simulink model "PV_twin_final"  (R2024b)
settings: Solver=ode23t  StartTime=0.0  StopTime=2  RelTol=1e-3
InitFcn:
  | Ts_Control = 10e-5;
  | Ts_Power = 80e-6;
  | Sensor_Ts = 1e-05;
libraries: spsSeriesRLCBranchLib x4, spsIGBTDiodeLib x4, spsCurrentMeasurementLib x2, spsVoltageMeasurementLib x2, spsACVoltageSourceLib x1, spsDiodeLib x1, spsIGBTLib x1, slpidlib x1, spsPVArrayLib x1, spsPWMGeneratorDCDCLib x1, simulink x1, spspowerguiLib x1
settings Model: SimulationMode=accelerator  Creator=Deependra  LastModifiedBy=Asus
settings DataIOCC: ReturnWorkspaceOutputs=off
settings DebuggingCC: UnconnectedInputMsg=warning  UnconnectedOutputMsg=warning  UnconnectedLineMsg=warning  ArithmeticOperatorsInVariantConditions=warning
settings ModelReferenceCC: EnableRefExpFcnMdlSchedulingChecks=on
settings SFSimCC: SimUseLocalCustomCode=off  CustomCodeUndefinedFunction=UseInterfaceOnly
settings RTWCC: RTWUseLocalCustomCode=off  GPUComputeCapability=3.5

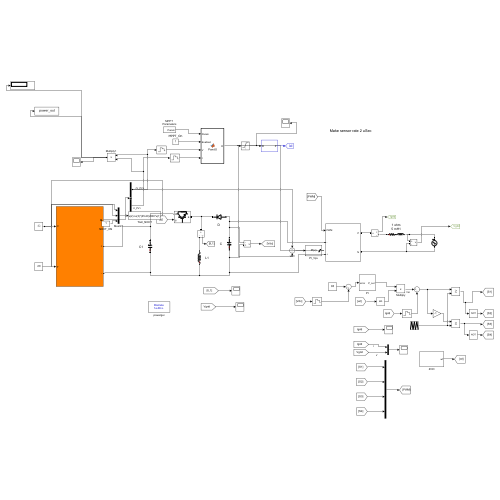
[thumbnail: Simulink's stored preview of the top-level diagram]
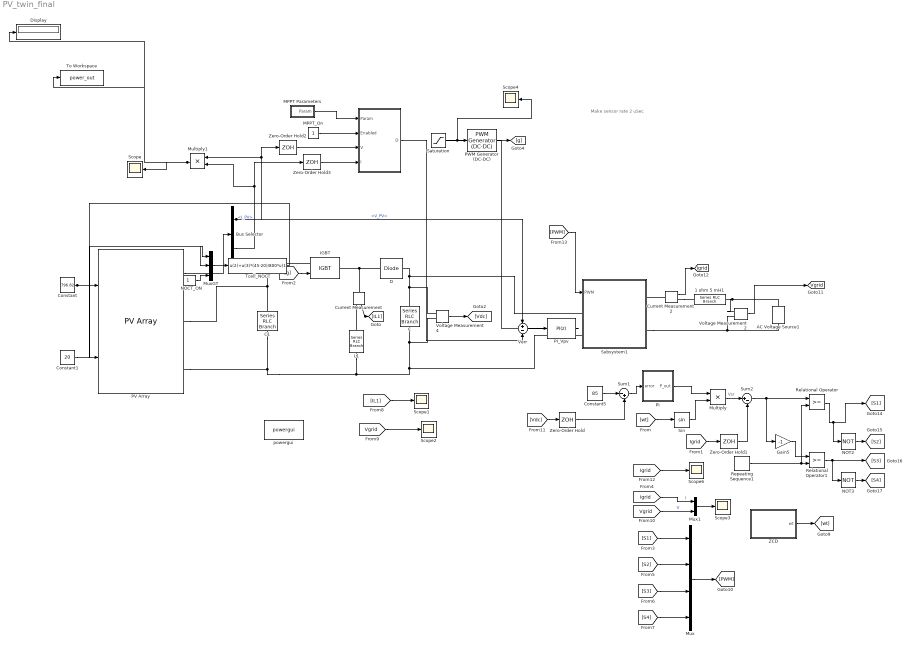
== system PV_twin_final ==
  note: Make sensor rate 2 uSec
  " " : MATLAB Function  TreatAsAtomicUnit=on
  1 ohm 5 mH1 : spsSeriesRLCBranchLib/Series RLC Branch  LConnTagsString=__new0  RConnTagsString=__new0  BranchType=RL  Resistance=1  Inductance=5e-3  SetiL0=off  InitialCurrent=0  Capacitance=400e-6  Setx0=off  InitialVoltage=0  Measurements=None
  AC Voltage Source1 : spsACVoltageSourceLib/AC Voltage Source  Amplitude=64  Phase=0  Frequency=50  SampleTime=0  Measurements=None  BusType=swing  Pref=10e3  Qref=0  Qmin=-inf  Qmax=+inf
  Bus Selector : BusSelector  OutputSignals=V_PV,I_PV
  C : spsSeriesRLCBranchLib/Series RLC Branch  LConnTagsString=__new0  RConnTagsString=__new0  BranchType=C  Resistance=1e-4  Inductance=200e-6  SetiL0=off  InitialCurrent=0  Capacitance=680e-6  Setx0=off  InitialVoltage=7.5  Measurements=None
  C1 : spsSeriesRLCBranchLib/Series RLC Branch  LConnTagsString=__new0  RConnTagsString=__new0  BranchType=C  Resistance=1e-4  Inductance=200e-6  SetiL0=off  InitialCurrent=0  Capacitance=680e-6  Setx0=off  InitialVoltage=7.5  Measurements=None
  Constant : Constant  Value=796.82
  Constant1 : Constant  Value=20
  Constant5 : Constant  Value=85
  Current Measurement : spsCurrentMeasurementLib/Current Measurement  PhasorSimulation=off  OutputType=Complex  PSBequivalent=0
  Current Measurement2 : spsCurrentMeasurementLib/Current Measurement  PhasorSimulation=off  OutputType=Complex  PSBequivalent=0
  "D " : spsDiodeLib/Diode  Ron=1e-3  Lon=0  Vf=0  IC=0  UseSnubber=off  Rs=inf  Cs=inf  Measurements=off
  Display : Display
  Gain5 : Gain  Gain=-1
  IGBT : spsIGBTLib/IGBT  Ron=0.000001  Lon=0  Vf=0  Tf=1e-6  Tt=2e-6  IC=0  Rs=1e5  Cs=inf  Measurements=off
  L1 : spsSeriesRLCBranchLib/Series RLC Branch  LConnTagsString=__new0  RConnTagsString=__new0  BranchType=L  Resistance=1e-4  Inductance=5e-3  SetiL0=off  InitialCurrent=14  Capacitance=30e-6  Setx0=off  InitialVoltage=150  Measurements=None
  MPPT Parameters : Subsystem
  MPPT_On : Constant
  Multiply : Product
  Multiply1 : Product
  Mux : Mux
  Mux1 : Mux  Inputs=2
  MuxGT : Mux  Inputs=3
  NOCT_ON : Constant
  NOT2 : Logic  Operator=NOT  AllPortsSameDT=off  OutDataTypeStr=boolean
  NOT3 : Logic  Operator=NOT  AllPortsSameDT=off  OutDataTypeStr=boolean
  PI : Subsystem
  PI_Vpv : slpidlib/PID Controller  Controller=PI  Form=Parallel  TimeDomain=Discrete-time  UseExternalTs=off  SampleTime=20e-6  IntegratorMethod=Forward Euler  FilterMethod=Forward Euler  ControllerParametersSource=internal  P=0.1  I=20  UseKiTs=off  D=0  UseExternalDerivativeSource=off  N=100  UseFilter=on  TunerSelectOption=Transfer Function Based (PID Tuner App)  InitialConditionSource=internal  InitialConditionForIntegrator=0.6  InitialConditionForFilter=0  DifferentiatorICPrevScaledInput=0  ExternalReset=none  TrackingMode=off  Kt=1  LimitOutput=on  SatLimitsSource=internal  UpperSaturationLimit=0.87  LowerSaturationLimit=0  LinearizeAsGain=off  AntiWindupMode=clamping  Kb=1  LimitIntegrator=off  UpperIntegratorSaturationLimit=inf  LowerIntegratorSaturationLimit=-inf  POutMin=[]  POutMax=[]  IOutMin=[]  IOutMax=[]  DOutMin=[]  DOutMax=[]  NOutMin=[]  NOutMax=[]  SumOutMin=[]  SumOutMax=[]  SaturationOutMin=[]  SaturationOutMax=[]  PParamMin=[]  PParamMax=[]  IParamMin=[]  IParamMax=[]  DParamMin=[]  DParamMax=[]  NParamMin=[]  NParamMax=[]  KbParamMin=[]  KbParamMax=[]  KtParamMin=[]  KtParamMax=[]  KbOutMin=[]  KbOutMax=[]  KtOutMin=[]  KtOutMax=[]  IntegratorOutMin=[]  IntegratorOutMax=[]  FilterOutMin=[]  FilterOutMax=[]  SumI1OutMin=[]  SumI1OutMax=[]  SumI2OutMin=[]  SumI2OutMax=[]  SumI3OutMin=[]  SumI3OutMax=[]  SumI4OutMin=[]  SumI4OutMax=[]  SumDOutMin=[]  SumDOutMax=[]  DifferentiatorOutMin=[]  DifferentiatorOutMax=[]  FilterDiffOutCoefMin=[]  FilterDiffOutCoefMax=[]  ReciprocalOutMin=[]  ReciprocalOutMax=[]  SumDenOutMin=[]  SumDenOutMax=[]  SumNumOutMin=[]  SumNumOutMax=[]  DivideOutMin=[]  DivideOutMax=[]  UdiffTsProdOutMin=[]  UdiffTsProdOutMax=[]  NTsProdOutMin=[]  NTsProdOutMax=[]  UintegralTsProdOutMin=[]  UintegralTsProdOutMax=[]  UngainTsProdOutMin=[]  UngainTsProdOutMax=[]  ClampingZeroOutDataTypeStr=Inherit: Inherit via back propagation  ClampingZeroOutMin=[]  ClampingZeroOutMax=[]  FilterDenConstantOutDataTypeStr=Inherit: Inherit via back propagation  FilterDenConstantOutMin=[]  FilterDenConstantOutMax=[]  PCopyOutDataTypeStr=Inherit: Inherit via back propagation  PCopyOutMin=[]  PCopyOutMax=[]  NCopyOutDataTypeStr=Inherit: Inherit via back propagation  NCopyOutMin=[]  NCopyOutMax=[]  IntegratorContinuousStateAttributes=''  IntegratorStateMustResolveToSignalObject=off  IntegratorRTWStateStorageClass=Auto  FilterContinuousStateAttributes=''  FilterStateMustResolveToSignalObject=off  FilterRTWStateStorageClass=Auto  ParallelPVariant=InternalParameters  IdealPVariant=Disabled  IVariant=InternalParameters  DVariant=Disabled  IntegratorVariant=Discrete  SatVariant=Enabled  AWVariant=DiscClampingParallel  PCopyVariant=Disabled  TRVariant=Disabled  FdbkBlocksVariant=Forward  IdealPFdbkVariant=Disabled  SatFdbkVariant=Disabled  DerivativeFilterVariant=Disabled  NVariant=Disabled  NCopyVariant=Disabled_SignalSpec  FilterICVariant=Disabled  IntegratorICVariant=InternalICs  ExternalResetVariant=Disabled  TRSumVariant=Passthrough  SumFdbkVariant=Disabled  SumVariant=Sum_PI  TsampFilterVariant=InternalTs  TsampNgainVariant=Passthrough  TsampIntegralVariant=Disabled_SignalSpec  ExternalSaturationOutDataTypeStr=Inherit: Same as second input  DerivativeSourceVariant=Disabled  PreIntVariant=InternalPreInt
      settings: LibrarySourceBlock=simulink/Discrete/Discrete PID Controller
  PV Array : spsPVArrayLib/PV Array  Npar=1  Nser=1  PlotType=one module @ 25 deg.C & specified irradiances  S_vec="[ 1000  500  100 ]"  Temp_C_vec="[ 45 25  ]"  ModuleName=User-defined  PlotWhenSelected=off  Pm=335.415  Ncell=72  Voc=46.27  Isc=9.41  Vm=37.9  Im=8.85  beta_Voc_pc=-0.30  alpha_Isc_pc=0.05  beta_Voc=-0.13881  alpha_Isc=0.004705  IL=9.4203  I0=3.2103e-11  nI=0.94785  Rsh=312.4283  Rs=0.34157  RobustModel=off  RobustCellTemperature=313.3991  BAL=off  Tc=1e-6  Tfilter=10e-5
  PWM Generator (DC-DC) : spsPWMGeneratorDCDCLib/PWM Generator (DC-DC)  Fsw=10e3  Ts=0
  Relational Operator : RelationalOperator  OutDataTypeStr=boolean  RndMeth=Simplest  InputSameDT=off
  Relational Operator1 : RelationalOperator  OutDataTypeStr=boolean  RndMeth=Simplest  InputSameDT=off
  Repeating Sequence1 : simulink/Sources/Repeating Sequence  rep_seq_t=[0 0.0001 0.0002]  rep_seq_y=[-1 1 -1]
  Saturation : Saturate  UpperLimit=0.87  LowerLimit=0
  Scope{,1..4,6} (6 alike) : Scope
  Sin : Trigonometry
  Subsystem1 : Subsystem
  Sum1 : Sum  Inputs=|-+
  Sum2 : Sum  Inputs=|+-
  Tcell_NOCT : Fcn  Expr=u(2)+u(3)*(45-20)/800*u(1)
  To Workspace : ToWorkspace  VariableName=power_out  SampleTime=-1
  Verr : Sum  Inputs=+-
  Voltage Measurement2 : spsVoltageMeasurementLib/Voltage Measurement  Tag=PoWeRsYsTeMmEaSuReMeNt  PhasorSimulation=off  OutputType=Magnitude  PSBequivalent=0
  Voltage Measurement4 : spsVoltageMeasurementLib/Voltage Measurement  PhasorSimulation=off  OutputType=Complex  PSBequivalent=0
  ZCD : Subsystem
  Zero-Order Hold : ZeroOrderHold  SampleTime=Sensor_Ts
  Zero-Order Hold1 : ZeroOrderHold  SampleTime=Sensor_Ts
  Zero-Order Hold2 : ZeroOrderHold  SampleTime=0.01
  Zero-Order Hold3 : ZeroOrderHold  SampleTime=0.01
  powergui : spspowerguiLib/powergui  Priority=1  SimulationMode=Discrete  SampleTime=1e-6  frequency=50  Iterations=50  frequencyindice=0  Pbase=100e6  ErrMax=1e-4  UnitsV=kV  UnitsW=MW  buscounter=0  FunctionMessages=off  echomessages=off  EnableUseOfTLC=off  CurrentSourceSwitches=off  DisableSnubberDevices=off  DisableRonSwitches=off  DisableVfSwitches=off  DisplayEquations=off  AutomaticDiscreteSolvers=off  SolverType=Tustin/Backward Euler (TBE)  Interpol=off  ExternalGateDelay=off  methode=off  Ts=100  x0status=blocks  SPID=on  SwTol=0  HookPort=off  NonlinearTolerance=1e-4  nMaxIteration=100  ContinueOnMaxIteration=off  RestoreLinks=warning  ResistiveCurrentMeasurement=off  Frange=[0:2:500]  Ylog=off  Xlog=on  ShowGrid=off  save=off  variable=ZData  structure=0  ZoomFFT=off  StartTime=0.0  cycles=1  DisplayStyle=1  fundamental=60  FreqAxis=off  MaxFrequency=1000  frequencyindicesteady=1  RmsSteady=1  display=off
  tag scope: Igrid=global, Vgrid=global
  wires:
  [g] -> IGBT/1
  Current Measurement/1 -> [IL1]
  Constant/1 -> PV Array/1, MuxGT/1
  PV Array/1 -> Bus Selector/1
  [Vdc] -> Zero-Order Hold/1
  Constant5/1 -> Sum1/1
  [wt] -> Sin/1
  Sin/1 -> Multiply/2
  Multiply/1 -> Sum2/1  "Vsr"
  [Igrid] -> Zero-Order Hold1/1
  ZCD/1(wt) -> [wt]
  [S2] -> Mux/2
  [S1] -> Mux/1
  [S3] -> Mux/3
  [S4] -> Mux/4
  Mux/1 -> [PWM]
  [IL1] -> Scope1/1
  [Vgrid] -> Scope2/1
  Voltage Measurement4/1 -> [Vdc]
  PWM Generator (DC-DC)/1 -> [g]
  MPPT_On/1 -> " "/2(Enabled)
  MPPT Parameters/1(Param) -> " "/1(Param)
  Bus Selector/1 -> Multiply1/1, Zero-Order Hold2/1, Verr/1  "<V_PV>"
  Bus Selector/2 -> Multiply1/2, Zero-Order Hold3/1  "<I_PV>"
  Saturation/1 -> Scope4/1, PWM Generator (DC-DC)/1
  Mux1/1 -> Scope3/1
  [Igrid] -> Mux1/1  "I"
  [Vgrid] -> Mux1/2  "V"
  Voltage Measurement2/1 -> [Vgrid]
  Current Measurement2/1 -> [Igrid]
  [PWM] -> Subsystem1/1(PWM)
  Relational Operator/1 -> NOT2/1, [S1]
  Repeating Sequence1/1 -> Relational Operator1/2, Relational Operator/2
  Relational Operator1/1 -> NOT3/1, [S3]
  NOT2/1 -> [S2]
  Sum2/1 -> Relational Operator/1, Gain5/1
  Gain5/1 -> Relational Operator1/1
  NOT3/1 -> [S4]
  [Igrid] -> Scope6/1
  Zero-Order Hold/1 -> Sum1/2
  Zero-Order Hold1/1 -> Sum2/2
  Sum1/1 -> PI/1(error)
  PI/1(P_out) -> Multiply/1
  Zero-Order Hold2/1 -> " "/3(V)
  Zero-Order Hold3/1 -> " "/4(I)
  Multiply1/1 -> Scope/1, To Workspace/1, Display/1
  " "/1(D) -> Verr/2
  Verr/1 -> PI_Vpv/1
  PI_Vpv/1 -> Saturation/1
  Constant1/1 -> MuxGT/2
  NOCT_ON/1 -> MuxGT/3
  MuxGT/1 -> Tcell_NOCT/1
  Tcell_NOCT/1 -> PV Array/2
  connections:
  C1/RConn1 -- PV Array/RConn1 -- IGBT/LConn1
  "D "/RConn1 -- Current Measurement/LConn1 -- IGBT/RConn1
  C/RConn1 -- Voltage Measurement4/LConn2 -- Subsystem1/LConn1 -- "D "/LConn1
  PV Array/RConn2 -- C1/LConn1 -- L1/LConn1 -- Subsystem1/LConn2 -- Voltage Measurement4/LConn1 -- C/LConn1
  L1/RConn1 -- Current Measurement/RConn1
  Voltage Measurement2/LConn1 -- 1 ohm 5 mH1/RConn1 -- AC Voltage Source1/RConn1
  Voltage Measurement2/LConn2 -- AC Voltage Source1/LConn1 -- Subsystem1/RConn2
  Current Measurement2/RConn1 -- 1 ohm 5 mH1/LConn1
  Current Measurement2/LConn1 -- Subsystem1/RConn1

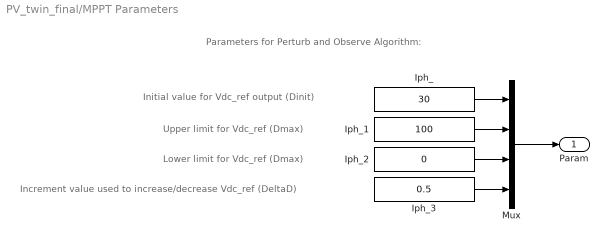
== system PV_twin_final/MPPT Parameters ==
  note: Parameters for Perturb and Observe Algorithm:
  note: Lower limit for Vdc_ref (Dmax)
  note: Initial value for Vdc_ref output (Dinit)
  note: Increment value used to increase/decrease Vdc_ref (DeltaD)
  note: Upper limit for Vdc_ref (Dmax)
  Iph_ : Constant  Value=30
  Iph_1 : Constant  Value=100
  Iph_2 : Constant  Value=0
  Iph_3 : Constant  Value=0.5
  Mux : Mux
  Param : Outport  VectorParamsAs1DForOutWhenUnconnected=off
  wires:
  Mux/1 -> Param/1
  Iph_3/1 -> Mux/4
  Iph_2/1 -> Mux/3
  Iph_1/1 -> Mux/2
  Iph_/1 -> Mux/1

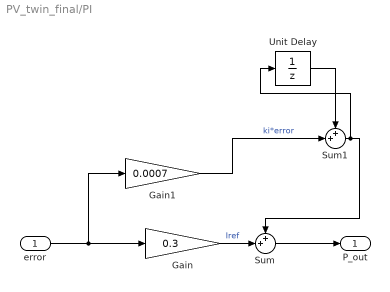
== system PV_twin_final/PI ==
  error : Inport
  Gain : Gain  Gain=0.3
  Gain1 : Gain  Gain=0.0007
  Sum : Sum  Inputs=++|
  Sum1 : Sum  Inputs=++|
  Unit Delay : UnitDelay  SampleTime=50e-6  HasFrameUpgradeWarning=on
  P_out : Outport  VectorParamsAs1DForOutWhenUnconnected=off
  wires:
  Gain/1 -> Sum/2  "Iref"
  error/1 -> Gain/1, Gain1/1
  Gain1/1 -> Sum1/2  "ki*error"
  Sum/1 -> P_out/1
  Unit Delay/1 -> Sum1/1
  Sum1/1 -> Sum/1, Unit Delay/1

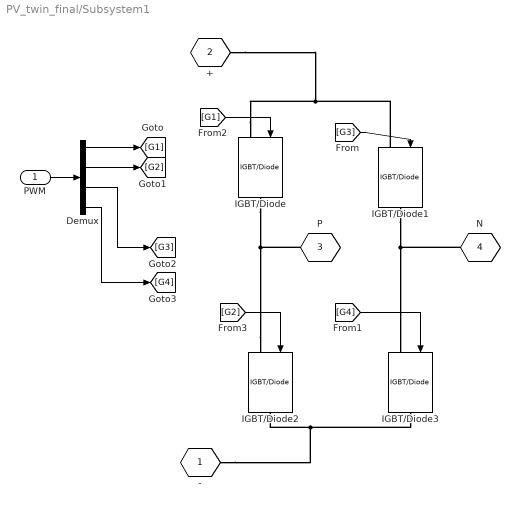
== system PV_twin_final/Subsystem1 ==
  PWM : Inport
  Demux : Demux
  IGBT/Diode{,1..3} (4 alike) : spsIGBTDiodeLib/IGBT//Diode  Ron=1e-3  Rs=1e5  Cs=inf  Measurements=off
  - : PMIOPort  Tag=PMCPort  Side=Left
  + : PMIOPort  Tag=PMCPort  Port=2  Side=Left
  "P " : PMIOPort  Tag=PMCPort  Port=3  Side=Right
  "N " : PMIOPort  Tag=PMCPort  Port=4  Side=Right
  wires:
  Demux/4 -> [G4]
  Demux/3 -> [G3]
  Demux/2 -> [G2]
  Demux/1 -> [G1]
  PWM/1 -> Demux/1
  [G4] -> IGBT/Diode3/1
  [G1] -> IGBT/Diode/1
  [G2] -> IGBT/Diode2/1
  [G3] -> IGBT/Diode1/1
  connections:
  IGBT/Diode/LConn1 -- +/RConn1 -- IGBT/Diode1/LConn1
  "N "/RConn1 -- IGBT/Diode3/LConn1 -- IGBT/Diode1/RConn1
  IGBT/Diode2/RConn1 -- -/RConn1 -- IGBT/Diode3/RConn1
  IGBT/Diode2/LConn1 -- "P "/RConn1 -- IGBT/Diode/RConn1

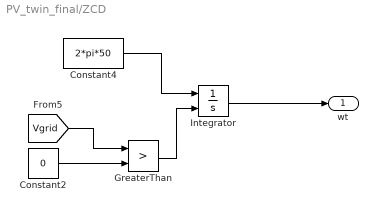
== system PV_twin_final/ZCD ==
  Constant2 : Constant  Value=0
  Constant4 : Constant  Value=2*pi*50
  GreaterThan : RelationalOperator  Operator=>  OutDataTypeStr=boolean  RndMeth=Simplest  InputSameDT=off
  Integrator : Integrator  ExternalReset=rising
  wt : Outport  VectorParamsAs1DForOutWhenUnconnected=off
  wires:
  Constant4/1 -> Integrator/1
  Integrator/1 -> wt/1
  [Vgrid] -> GreaterThan/1
  GreaterThan/1 -> Integrator/2
  Constant2/1 -> GreaterThan/2

== matlab function PV_twin_final/  ==
  settings: updateMethod=DISCRETE  sampleTime=Ts_Control
  data: Param input; Enabled input; V input; I input; D output
function D  = PandO(Param, Enabled, V, I)

% MPPT controller based on the Perturb & Observe algorithm.

% D output = Reference for DC link voltage (Vdc_ref) 
%
% Enabled input = 1 to enable the MPPT controller
% V input = PV array terminal voltage (V)
% I input = PV array current (A)
%
% Param input:
Dinit = Param(1);  %Initial value for Vdc_ref
Dmax = Param(2);   %Maximum value for Vdc_ref
Dmin = Param(3);   %Minimum value for Vdc_ref
deltaD = Param(4); %Increment value used to increase/decrease Vdc_ref
%  

persistent Vold Pold Dold;

dataType = 'double';

if isempty(Vold)
    Vold=0;
    Pold=0;
    Dold=Dinit;
end
P= V*I;
dV= V - Vold;
dP= P - Pold;

if dP ~= 0 & Enabled ~=0
    if dP < 0
        if dV < 0
            D = Dold + deltaD;
        else
            D = Dold - deltaD;
        end
    else
        if dV < 0
            D = Dold - deltaD;
        else
            D = Dold + deltaD;
        end    
    end
else D=Dold;
end

if D >= Dmax | D<= Dmin
    D=Dold;
end

Dold=D;
Vold=V;
Pold=P;
